simulink model "roll_model_TRUCKSIM_18DOF_REVISED"  (R2023b)
settings: Solver=FixedStepAuto  StartTime=0.0  StopTime=20  FixedStep=0.0005  RelTol=1e-3
StopFcn:
  | save_dataset_18state;
libraries: Solver_SF x1
(part 5 of 5)

== matlab function roll_model_TRUCKSIM_18DOF_REVISED/Subsystem2/MATLAB Function2 ==
  settings: updateMethod=DISCRETE
  data: delta_cmd input; u9 output; Mact_cmd input; Fx_req input; x input; omega_ref input; Fz6 input; Fy6 input; mu_road input; u_prev input; Tb_base output; Tb_wheel output; rho output; alloc_diag output
function [u9,Tb_base,Tb_wheel,rho,alloc_diag] = ...
    fcn(delta_cmd,Mact_cmd,Fx_req,x,omega_ref,Fz6,Fy6,mu_road,u_prev)
%#codegen
% =========================================================================
% BLOCK 3 - LEGACY RULE-BASED ALLOCATION + ACTUATOR PACK
% DLC11 speed-loop candidate 2026-11-24; untouched active-roll command
% SMOOTH BRAKE + SINGLE-STAGE ACTIVE ROLL COMMAND
%
% Keeps:
%   Tdrive_max = 20000 Nm
%   Tb_max     = 20000 Nm
%   traction allocation = common FRONT drive torque
%   braking allocation  = 35% front / 40% tractor rear / 25% trailer
%   L/R base split      = 50/50
%   Tdrive LPF tau_T    = 0.9 s
%   Tdrive_rate         = 9000 Nm/s
%   Tb_rate (apply)     = 4000 Nm/s
%   Tb_rate (release)   = 5000 Nm/s
%   Komega              = 60
%   phi_omega           = 4
%   omega_dead          = 1
%
% Main smoothing changes:
%   1) Removes hard front-brake clamp to exactly 50 Nm.
%   2) Applies first-order smoothing to brake target before slew limiting.
%   3) Uses asymmetric brake slew: normal apply, slightly faster release.
%   4) Prevents DRIVE and new brake target from being commanded together.
%   5) Keeps all main speed-tracking parameters unchanged.
%   6) Passes through signed Mact_cmd already rate-limited in Block 2.
% =========================================================================

Ts = 0.01;

% R25 U4 BRAKE SMOOTHING A/B -- ONLY BLOCK 3; NO CHANGE TO U2 CONTROL
% 0 = exact original brake filter / wheel SMC values
% 1 = gentler brake-target LPF only (first test)
% 2 = mode 1 + milder wheel-speed SMC brake correction (second test)
% These changes are diagnostic, not TruckSim-validated.
brakeSmoothMode = 2.0;

% ================================================================
% DRIVE RIPPLE REDUCTION - REAL ACTUATOR COMMAND, NOT alloc_diag
% 0 = EXACT original u9(2) logic in this uploaded Block 3 (baseline)
% 1 = prior mild smoothing, near speed reference (kept for comparison)
% 2 = NEW continuous two-stage low-pass throughout DRIVE, adaptive to speed
%     error. No abrupt abs(ev_guard)<0.30 enable/disable boundary.
% 3 = ULTRA mode (more filtering; can degrade speed tracking)
% NOTE: COAST/BRAKE retain fast torque release for safety.
% ================================================================
driveSmoothMode = 2.0; % DLC diagnostic: reduce actuator delay

%% Fixed-size outputs
u9         = zeros(9,1);
Tb_base    = zeros(6,1);
Tb_wheel   = zeros(6,1);
rho        = zeros(6,1);
alloc_diag = zeros(5,1);

%% Vehicle parameters
Rf = 0.51;
Rr = 0.51;
Rs = 0.51;

omega = [x(9);x(10);x(11);x(12);x(13);x(14)];

%% KEEP THESE VALUES - THEY ARE CURRENTLY GIVING GOOD SPEED TRACKING
Tdrive_max = 20000.0;
Tb_max     = 20000.0;

%% ========================================================================
% ROAD-AWARE AVAILABLE LONGITUDINAL FORCE
% ========================================================================

mu_eff = clamp(mu_road,0.10,1.20);

Fx_cap = zeros(6,1);

for i = 1:6
    Fz_i = max(Fz6(i),1.0);

    c2 = (mu_eff*Fz_i)^2 - Fy6(i)^2;

    if c2 > 0.0
        Fx_cap(i) = sqrt(c2);
    else
        Fx_cap(i) = 0.0;
    end
end

Fx_req_raw = Fx_req;

%% ========================================================================
% TRACTION / BRAKING CAPACITY
% ========================================================================

traction_util = 0.97; %#ok<NASGU>
brake_util    = 0.90;

% Keep the user's current setting: motor limit is the traction cap.
Fdrive_motor_cap = Tdrive_max/Rf;
Fdrive_cap       = Fdrive_motor_cap;

Fbrake_cap = brake_util*sum(Fx_cap);

if Fx_req_raw >= 0.0
    Fx_req_lim = min(Fx_req_raw,Fdrive_cap);
else
    Fx_req_lim = max(Fx_req_raw,-Fbrake_cap);
end

%% ========================================================================
% DRIVE / COAST / BRAKE HYSTERESIS
% ========================================================================

Fx_drive_on  =   900.0;  % below nominal steady force (~2232 N)
Fx_drive_off =   200.0;
Fx_brake_on  = -1500.0;
Fx_brake_off =  -400.0;

prevDrive = (u_prev(2) > 200.0);

prevBrakeTorque = ...
      u_prev(4)+u_prev(5) ...
    + u_prev(6)+u_prev(7) ...
    + u_prev(8)+u_prev(9);

prevBrake = (prevBrakeTorque > 200.0);

mode = 0.0;

if prevDrive

    if Fx_req_lim >= Fx_drive_off
        mode = 1.0;
    elseif Fx_req_lim <= Fx_brake_on
        mode = -1.0;
    else
        mode = 0.0;
    end

elseif prevBrake

    if Fx_req_lim <= Fx_brake_off
        mode = -1.0;
    elseif Fx_req_lim >= Fx_drive_on
        mode = 1.0;
    else
        mode = 0.0;
    end

else

    if Fx_req_lim >= Fx_drive_on
        mode = 1.0;
    elseif Fx_req_lim <= Fx_brake_on
        mode = -1.0;
    else
        mode = 0.0;
    end

end

%% ========================================================================
% R25 A/B DIAGNOSTIC - SPEED-ERROR DRIVE/BRAKE GUARD
% Only enable for scenario 8/9 (same test speed reference).
% The rear-axle wheel references in Block 2 are:
%  omega_ref(3)=(vx_ref-rt_ref*Tr/2)/Rr
%  omega_ref(4)=(vx_ref+rt_ref*Tr/2)/Rr
% so their mean reconstructs vx_ref for forward motion.
%
% speedGuardTest = 0 : exact previous fast-release-test behavior
% speedGuardTest = 1 : prevent continued braking when already underspeed
% Set to 0 again for legacy scenarios (1-6).
% ========================================================================
speedGuardTest = 1.0;
vx_ref_est = 0.5*Rr*(max(omega_ref(3),0.0)+max(omega_ref(4),0.0));
ev_guard = x(1)-vx_ref_est;  % positive = actual vehicle too fast

if speedGuardTest > 0.5
    if ev_guard < -0.35
        % Below speed target: BRAKE is never allowed to persist.
        % Drive only if Block 2 explicitly requests positive force.
        if Fx_req_lim > Fx_drive_off
            mode = 1.0;
        else
            mode = 0.0;
        end
    elseif ev_guard > 0.60 && mode > 0.5
        % Above target: do not keep applying power, even if a stale positive
        % model-assisted request remains. Let force controller decide BRAKE
        % on a later sample; do not force large unrequested brake torques.
        mode = 0.0;
    end
end

%% ========================================================================
% LEGACY RULE-BASED LONGITUDINAL ALLOCATION
% ========================================================================

Tdrive_target = 0.0;

if mode > 0.5

    % DRIVE
    Fx_drive_cmd = max(Fx_req_lim,0.0);

    Tdrive_target = Fx_drive_cmd*Rf;
    Tdrive_target = clamp(Tdrive_target,0.0,Tdrive_max);

    Tb_base(:) = 0.0;

elseif mode < -0.5

    % BRAKE
    Tdrive_target = 0.0;

    Fb = max(-Fx_req_lim,0.0);

    wf = 0.35;
    wr = 0.40;
    ws = 0.25;

    Fbf = 0.5*wf*Fb;
    Fbr = 0.5*wr*Fb;
    Fbs = 0.5*ws*Fb;

    %% Symmetric L/R axle capacity
capFront = min( ...
    min(Fx_cap(1),Fx_cap(2)), ...
    Tb_max/Rf);

capRear = min( ...
    min(Fx_cap(3),Fx_cap(4)), ...
    Tb_max/Rr);

capTrailer = min( ...
    min(Fx_cap(5),Fx_cap(6)), ...
    Tb_max/Rs);

%% Preserve 50/50 L/R allocation
Fbf_each = min(Fbf,capFront);
Fbr_each = min(Fbr,capRear);
Fbs_each = min(Fbs,capTrailer);

FbfL = Fbf_each;
FbfR = Fbf_each;

FbrL = Fbr_each;
FbrR = Fbr_each;

FbsL = Fbs_each;
FbsR = Fbs_each;

    Tb_base(1) = FbfL*Rf;
    Tb_base(2) = FbfR*Rf;

    Tb_base(3) = FbrL*Rr;
    Tb_base(4) = FbrR*Rr;

    Tb_base(5) = FbsL*Rs;
    Tb_base(6) = FbsR*Rs;

else

    % COAST
    Tdrive_target = 0.0;
    Tb_base(:) = 0.0;

end

%% ========================================================================
% WHEEL-SPEED SMC BRAKE CORRECTION
%
% KEEP USER'S CURRENT GAINS.
% Only active in BRAKE mode so it cannot fight traction.
% ========================================================================

Komega     = 60.0;
phi_omega  = 4.0;
omega_dead = 1.0;

if brakeSmoothMode > 1.5
    % More gentle brake wheel-speed correction. Do not change the
    % normal base allocation 35/40/25, motor, or speed guard.
    Komega    = 40.0;
    phi_omega = 6.0;
end

if mode < -0.5

    for i = 1:6

        ew = omega(i)-omega_ref(i);

        if ew > omega_dead
            z = (ew-omega_dead)/phi_omega;
            Tb_wheel(i) = Komega*satfun(z);
        else
            Tb_wheel(i) = 0.0;
        end

    end

else

    Tb_wheel(:) = 0.0;

end

%% ========================================================================
% RAW BRAKE TARGET
% ========================================================================

Tb_target_raw = zeros(6,1);

for i = 1:6

    Tb_target_raw(i) = clamp( ...
        Tb_base(i)+Tb_wheel(i), ...
        0.0, ...
        Tb_max);

end

%% ========================================================================
% DRIVE TORQUE SMOOTHING
%
% KEEP CURRENT VALUES because they are giving good vx tracking.
% ========================================================================

% ================================================================
% R25 LONGITUDINAL A/B TEST: FAST RELEASE OF RESIDUAL DRIVE TORQUE
%
% 0: Original behavior, exact parity with the original Block 3.
% 1: During a confirmed BRAKE request, reduce DRIVE torque faster.
%    All brake allocation, friction limits, steering, active roll,
%    wheel SMC, and diagnostic filters are UNCHANGED.
%
% WHY: with tau_T=0.9 s the front-brake interlock below keeps the
% front brake from increasing until residual drive torque falls below
% 300 Nm. From 8000 Nm, this can take ~3 seconds. For the R25 entry
% transition (~2.2 seconds), the brakes may arrive much too late.
% ================================================================
fastDriveReleaseTest = 1.0;

% OPTIONAL A/B TEST B (only after evaluating Block 2 fine tune):
% 0 = original overspeed release threshold 0.45 m/s
% 1 = release residual drive at 0.30 m/s overspeed
R25_overspeedReleaseTest = 0.0;
overspeedReleaseThreshold = 0.45;
if R25_overspeedReleaseTest > 0.5
    overspeedReleaseThreshold = 0.30;
end

tau_T = 0.9;
Tdrive_rate = 9000.0;
if fastDriveReleaseTest > 0.5 && mode < -0.5
    tau_T = 0.2;          % fast drive release on BRAKE
    Tdrive_rate = 24000.0;
end

if speedGuardTest > 0.5
    if ev_guard > overspeedReleaseThreshold && mode < 0.5
        % Vehicle overspeed: remove residual DRIVE torque promptly.
        tau_T = 0.12;
        Tdrive_rate = 24000.0;
    elseif ev_guard < -0.35 && mode > 0.5
        % Underspeed: moderate drive build-up (no instantaneous torque).
        tau_T = 0.35;
    end
end

% ========================================================================
% R25 TEST C - EARLY DRIVE RELEASE (A/B)
% 0 = original Block 3 behavior; 1 = faster reduction of residual drive.
% No extra inputs/outputs. For scenarios 1-6, restore this switch to 0.
% ========================================================================
earlyDriveReleaseTest = 1.0;
if earlyDriveReleaseTest > 0.5
    if driveSmoothMode < 0.5
        % A/B baseline: original behavior, including fast release while DRIVE.
        releaseRequested = (mode < 0.5) || ...
            (ev_guard > -0.35 && Tdrive_target < u_prev(2)-150.0);
    else
        % The old 150-Nm rule also switched tau_T to 0.18 s during DRIVE,
        % making u9(2) follow oscillatory Fx_req too quickly.
        % Keep rapid actuator release ONLY in COAST or BRAKE.
        releaseRequested = (mode < 0.5);
    end
    if releaseRequested
        tau_T = min(tau_T,0.18);
        Tdrive_rate = max(Tdrive_rate,24000.0);
    end
end

% ================================================================
% R25 REAL DRIVE TORQUE SMOOTHING (u9(2) ACTUAL COMMAND)
%
% The old Mode 2 only ran when abs(ev_guard)<0.30. Crossing this limit
% repeatedly switched tau_T between fast/slow values, which can leave
% visible ripple even with a very large tau_T near the speed reference.
%
% New modes 2/3 use TWO cascaded low-pass stages in DRIVE:
%     requested torque -> driveTargetLP -> u_prev(2) -> u9(2)
% The first stage is persistent; the second is the existing actuator LPF.
% A smooth speed-error weight avoids an abrupt filtering-mode boundary.
%
% When the vehicle is far BELOW vx_ref, both filters speed up to preserve
% acceleration. On COAST/BRAKE, reset the target filter and retain the
% existing fast release (no torque hold through a braking request).
% These are candidate tuning values; compare actual vx/torque in TruckSim.
% ================================================================

persistent driveTargetLP;
if isempty(driveTargetLP)
    driveTargetLP = 0.0;
end

Tdrive_target_for_LPF = Tdrive_target;

if driveSmoothMode > 1.5 && mode > 0.5

    % Continuous smooth transition: below reference -> quick throttle;
    % near reference -> strong smoothing. No abs(ev_guard) mode jump.
    wSmooth = clamp((ev_guard+0.60)/0.55,0.0,1.0);
    wSmooth = wSmooth*wSmooth*(3.0-2.0*wSmooth);

    if driveSmoothMode < 2.5
        % MODE 2: strong but still intended for closed-loop control.
        tau_target_quiet = 0.10;   % [s] DLC: reduce phase lag
        tau_drive_quiet  = 0.30;   % [s] DLC: reduce second-stage delay
        rate_drive_quiet = 12000.0; % [Nm/s] quicker torque release/build-up
    else
        % MODE 3: ultra smooth, TEST ONLY (may add excessive delay).
        tau_target_quiet = 0.75;
        tau_drive_quiet  = 1.75;
        rate_drive_quiet = 2800.0;
    end

    % Preserve the response to a large vehicle underspeed.
    tau_target_fast = 0.06;
    tau_drive_fast  = 0.22;
    rate_drive_fast = 12000.0;

    tau_target = tau_target_fast + ...
        wSmooth*(tau_target_quiet-tau_target_fast);
    tau_T = tau_drive_fast + ...
        wSmooth*(tau_drive_quiet-tau_drive_fast);
    Tdrive_rate = rate_drive_fast + ...
        wSmooth*(rate_drive_quiet-rate_drive_fast);

    % When overspeed is developing and target torque is falling, do not
    % let the extra LPF continue to hold high residual driving torque.
    if ev_guard > 0.10 && Tdrive_target < u_prev(2)-150.0
        tau_target = min(tau_target,0.12);
        tau_T = min(tau_T,0.35);
        Tdrive_rate = max(Tdrive_rate,9000.0);
    end

    % Prefilter remains active on *every* DRIVE sample.
    a_target = Ts/(tau_target+Ts);
    driveTargetLP = driveTargetLP + ...
        a_target*(Tdrive_target-driveTargetLP);
    driveTargetLP = clamp(driveTargetLP,0.0,Tdrive_max);
    Tdrive_target_for_LPF = driveTargetLP;

elseif driveSmoothMode > 0.5 && driveSmoothMode < 1.5 && ...
       mode > 0.5 && abs(ev_guard) < 0.30 && ...
       Tdrive_target > 200.0

    % MODE 1: preserve the previous mild experiment exactly.
    tau_T = max(tau_T,1.50);
    Tdrive_rate = min(Tdrive_rate,5500.0);
    driveTargetLP = u_prev(2);

else
    % Outside DRIVE, do not keep an obsolete positive torque prefilter.
    % In Mode 0 this state is unused and original torque output is exact.
    if mode < 0.5
        driveTargetLP = 0.0;
    else
        driveTargetLP = u_prev(2);
    end
end

alpha_T = Ts/(tau_T+Ts);
Tdrive_target_f = ...
    u_prev(2) ...
    + alpha_T*(Tdrive_target_for_LPF-u_prev(2));

Tdrive = rate_limit( ...
    Tdrive_target_f, ...
    u_prev(2), ...
    Tdrive_rate*Ts);

Tdrive = clamp(Tdrive,0.0,Tdrive_max);

%% ========================================================================
% SMOOTH BRAKE TARGET
%
% THIS is the main new anti-chatter layer.
%
% tau_B controls brake smoothness:
%   smaller -> faster response
%   larger  -> smoother response
%
% Start at 0.12 s. It is short enough not to destroy speed tracking but
% removes the square pulses seen in U4/U6.
% ========================================================================

tau_B = 0.85;
if brakeSmoothMode > 0.5
    % Use only a modestly slower brake target filter to reduce ripples.
    % Keep fast underspeed brake RELEASE logic below unchanged.
    tau_B = 0.85;
end
if speedGuardTest > 0.5 && ev_guard < -0.35
    % As soon as the vehicle is too slow, release residual brakes quickly.
    % In particular, do not let BRAKE inertia persist through the acceleration
    % phase of the R25 reference. Brake torque still passes the rate limiter.
    tau_B = 0.435;
end
alpha_B = Ts/(tau_B+Ts);

Tb_target_f = zeros(6,1);

for i = 1:6

    Tb_target_f(i) = ...
        u_prev(3+i) ...
        + alpha_B*(Tb_target_raw(i)-u_prev(3+i));

end

%% ========================================================================
% BRAKE ACTUATOR SLEW LIMIT
%
% Keep nominal Tb_rate = 8000 Nm/s for application.
% Release is slightly faster so brakes do not drag when controller switches
% back toward coast/drive.
% ========================================================================

Tb_rate      = 4000.0;
Tb_rate_down = 5000.0;
if speedGuardTest > 0.5 && ev_guard < -0.35
    % Higher RELEASE rate only; never increase apply rate or brake cap.
    Tb_rate_down = 18000.0;
end

Tb = zeros(6,1);

for i = 1:6

    if Tb_target_f(i) >= u_prev(3+i)
        max_step = Tb_rate*Ts;
    else
        max_step = Tb_rate_down*Ts;
    end

    Tb(i) = rate_limit( ...
        Tb_target_f(i), ...
        u_prev(3+i), ...
        max_step);

    Tb(i) = clamp(Tb(i),0.0,Tb_max);

end

%% ========================================================================
% DRIVE/BRAKE INTERLOCK - SMOOTH VERSION
%
% IMPORTANT:
% The old code did:
%
%   if Tdrive > 300
%       Tb(1)=min(Tb(1),50)
%       Tb(2)=min(Tb(2),50)
%   end
%
% That directly created the 0 <-> 50 Nm square pulses in U4/U5.
%
% It is deliberately REMOVED.
%
% New logic only prevents NEW front brake demand during DRIVE; existing
% residual brake decays naturally through the LPF + release slew.
% ========================================================================

if Tdrive > 300.0

    % Do not create any new front-brake demand while driving.
    % Let existing residual front brake decay smoothly.
    for i = 1:2

        if Tb(i) > u_prev(3+i)
            Tb(i) = u_prev(3+i);
        end

    end

end

%% ========================================================================
% ACTIVE ROLL ACTUATOR - SINGLE-STAGE COMMAND (u9(3))
%
% The existing Block 2 already computes Mact_cmd with:
%   Mmax = 15000 Nm
%   MactRateMax = 15000 Nm/s
%   Mact_cmd = rate_limit(Mtarget,u_prev(3),MactRateMax*Ts)
%
% Do not add another LPF/rate limiter here. With the former tau_Mact=0.9 s
% and Ts=0.01 s, Block 3 passed only ~1.1% of each Block 2 increment.
% The resulting physical active-roll command was severely attenuated.
%
% Preserve the signed moment and exactly follow the Block 2 command.
% ========================================================================

Mact = Mact_cmd;

%% ========================================================================
% FINAL PHYSICAL COMMAND
% ========================================================================

u9(1) = delta_cmd;
u9(2) = Tdrive;
u9(3) = Mact;

u9(4) = Tb(1);
u9(5) = Tb(2);

u9(6) = Tb(3);
u9(7) = Tb(4);

u9(8) = Tb(5);
u9(9) = Tb(6);

% 3. Tính toán hệ số sử dụng lốp maxRho
Fx = zeros(6,1);
Fd = Tdrive / (2.0 * Rf);
Fx(1) =  Fd - Tb(1)/Rf;
Fx(2) =  Fd - Tb(2)/Rf;
Fx(3) = -Tb(3)/Rr;
Fx(4) = -Tb(4)/Rr;
Fx(5) = -Tb(5)/Rs;
Fx(6) = -Tb(6)/Rs;

maxRho_instant = 0.0; 
for i = 1:6
    Fz_i = max(Fz6(i), 100.0);
    den = mu_eff * Fz_i;
    
    if den > 1.0
        rho_i = sqrt(Fx(i)^2 + Fy6(i)^2) / den;
    else
        rho_i = 0.0;
    end
    
    if rho_i > maxRho_instant
        maxRho_instant = rho_i;
    end
end

% Dùng hàm tanh để bão hòa mượt, giúp đỉnh không bị phẳng lì hình chữ nhật
% Khi maxRho_instant tiến sát hoặc vượt 1.0, hàm tanh sẽ uốn cong mượt mà tiệm cận 1.0
maxRho_smooth = tanh(1.8 * maxRho_instant); 

% Lọc thông thấp với tau_rho lớn hơn để vê tròn hoàn toàn
persistent maxRho_filtered;
if isempty(maxRho_filtered)
    maxRho_filtered = 0.0;
end

tau_rho = 0.8;  % Tăng thời gian lọc lên 0.2 giây để làm mượt các vùng đỉnh
alpha_rho = Ts / (tau_rho + Ts);
maxRho_filtered = maxRho_filtered + alpha_rho * (maxRho_smooth - maxRho_filtered);

% Gán trực tiếp giá trị đã bão hòa mượt vào maxRho
maxRho = maxRho_filtered;
%% ========================================================================
% LỌC THÔNG THẤP CHO CÁC TÍN HIỆU ALLOC_DIAG ĐỂ TRÁNH GIẬT
% ========================================================================
persistent diag_filtered;
if isempty(diag_filtered)
    diag_filtered = zeros(5,1);
end

% Mảng chứa các giá trị thô trước khi lọc
alloc_diag_raw = zeros(5,1);
alloc_diag_raw(1) = Fx_req_raw;
alloc_diag_raw(2) = Fx_req_lim;       
alloc_diag_raw(3) = Tdrive;           % Dùng Tdrive đã qua bộ lọc cơ cấu chấp hành
alloc_diag_raw(4) = sum(Tb_target_raw);
alloc_diag_raw(5) = maxRho;           

% Hằng số thời gian lọc 
tau_diag = 0.7; 
alpha_diag = Ts / (tau_diag + Ts);

for k = 1:5
    if k ~= 5 
        diag_filtered(k) = diag_filtered(k) + alpha_diag * (alloc_diag_raw(k) - diag_filtered(k));
        alloc_diag(k) = diag_filtered(k);
    else
        alloc_diag(5) = maxRho; 
    end
end

%% ========================================================================
% OPTIONAL SECOND-STAGE FILTER FOR DISPLAY OF alloc_diag(2) ONLY
% IMPORTANT: alloc_diag(2) is a diagnostic; do NOT feed this filtered
% signal into Block 2/3 control loops or use it to claim reduced Fx_req
% chattering. The actual Fx_req_lim, u9, brakes and drive are unchanged.
%
% 0.0 = EXACT original alloc_diag(2) behavior (single LPF tau_diag=0.7 s)
% 1.0 = two-stage display-only LPF for easier Scope readability
% ========================================================================
diag2DisplaySmoothTest = 1.0;
tau_diag2_display = 3.0;     % [s] extra smoothing, adjust 0.6 ... 1.5

persistent diag2_display_state;
if isempty(diag2_display_state)
    diag2_display_state = 0.0;
end
if diag2DisplaySmoothTest > 0.5
    a2 = Ts/(tau_diag2_display+Ts);
    diag2_display_state = diag2_display_state + ...
        a2*(diag_filtered(2)-diag2_display_state);
    alloc_diag(2) = diag2_display_state;
else
    % Pass-through of the original already-filtered diagnostic.
    diag2_display_state = diag_filtered(2);
end

end % <--- KẾT THÚC HÀM TẠI ĐÂY (TUYỆT ĐỐI KHÔNG CÒN ĐOẠN GÁN GÌ NỮA)



function y = satfun(z)
%#codegen

if z > 1.0
    y = 1.0;
elseif z < -1.0
    y = -1.0;
else
    y = z;
end

end


function y = rate_limit(target,previous,max_step)
%#codegen

d = target-previous;

if d > max_step
    d = max_step;
elseif d < -max_step
    d = -max_step;
end

y = previous+d;

end


function y = clamp(x,lo,hi)
%#codegen

if x > hi
    y = hi;
elseif x < lo
    y = lo;
else
    y = x;
end

end
